simulink model "Finally_BPSK_Passband"  (R2026a)
settings: Solver=VariableStepDiscrete  StopTime=0.02  EnableMultiTasking=on
InitFcn:
  | commpassbandmodParams.Fc = 2.5e6;
  | commpassbandmodParams.F1 = commpassbandmodParams.Fc/3+.5e5;
libraries: commdigbbndpm3 x2, simulink x2, commfilt2 x2, commchan3 x1, commsink2 x1, dspsrcs4 x1, commrandsrc3 x1
Description:
  | Passband Modulation
  | 
  | This model shows a straightforward way to perform passband modulation, by multiplying a modulated complex signal with a complex sine wave to perform frequency upconversion.
settings Model: Creator=The MathWorks, Inc.  LastModifiedBy=MADHAV
settings SolverCC: InsertRTBMode=Auto
settings OptimizationCC: InitFltsAndDblsToZero=on  EfficientMapNaN2IntZero=off
settings DebuggingCC: SubsystemReferenceDiagnosticForUnitTest=warning
settings HardwareCC: ProdHWDeviceType=32-bit Generic
settings GRTTargetCC: CombineOutputUpdateFcns=off  GRTInterface=on

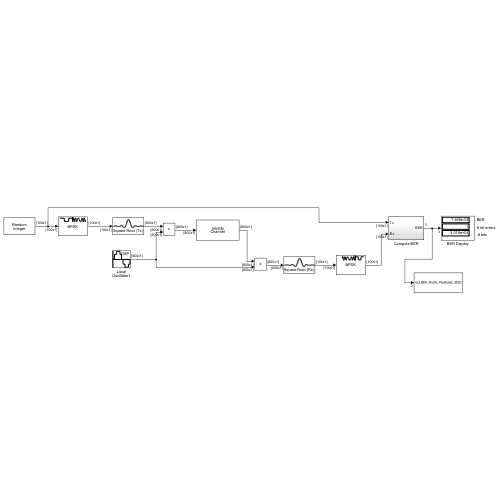
[thumbnail: Simulink's stored preview of the top-level diagram]
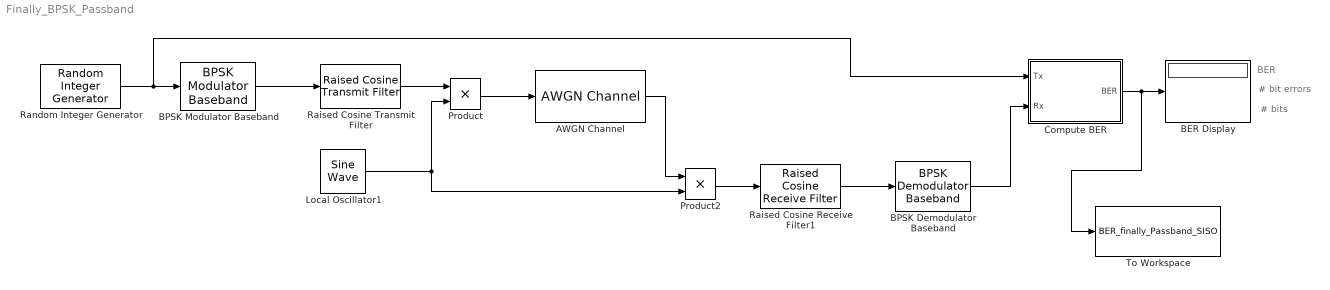
== system Finally_BPSK_Passband ==
  note: BER
  note: # bit errors
  note: # bits
  AWGN Channel : commchan3/AWGN Channel  LegacyMode=off  NoiseMethod="Signal to noise ratio  (SNR)"  noiseMode="Signal to noise ratio  (SNR)"  EbNo=10  EsNo=10  SNR=snr_variable  BitsPerSymbol=1  SignalPower=1  SpecifySymbolPeriod=off  SamplesPerSymbol=1  SymbolPeriod=1  VarianceSource=Parameter  Variance=1  RandomStream=Global stream  Seed=67  SimulateUsing=Code generation
  BER Display : Display
  BPSK Demodulator Baseband : commdigbbndpm3/BPSK Demodulator Baseband  DecType=Hard decision  VarSource=Dialog  Variance=1  Ph=0  outDtype=Inherit via internal rule  derotateFactorWordLen=16  derotateFactorDataTypeStr=Inherit: Same word length as input  derotateFactorLastDataTypeStr=Inherit: Same word length as input
      settings: LibrarySourceBlock=|
      | commhdldigbbndpm/BPSK
      | Demodulator
      | Baseband
  BPSK Modulator Baseband : commdigbbndpm3/BPSK Modulator Baseband  Ph=0  outDtype=double  outWordLen=16  outUDDataType=sfix(16)  outFracLenMode=Best precision  outFracLen=15  outDataTypeStr=double  outLastDataTypeStr=double
      settings: LibrarySourceBlock=|
      | commhdldigbbndpm/BPSK
      | Modulator
      | Baseband
  Compute BER : Subsystem
  Local Oscillator1 : dspsrcs4/Sine Wave  Amplitude=sqrt(2)  Frequency=commpassbandmodParams.Fc  Phase=0  SampleMode=Discrete  OutComplex=Real  CompMethod=Trigonometric fcn  TableSize=Speed  SampleTime=(1e-6) /8  SamplesPerFrame=800  ResetState=Restart at time zero  OutputFrames=off  dataType=double  wordLen=16  udDataType=sfix(16)  fracBitsMode=Best precision  numFracBits=15  OutDataTypeStr=double  LastOutDataTypeStr=double
  Product : Product  RndMeth=Zero
  Product2 : Product
  Raised Cosine Receive Filter1 : commfilt2/Raised Cosine Receive Filter  filtType=Square root  R=0.2  filtSpan=8  N=8  downFactor=8  downOffset=0  filterGain=2  InputProcessing=Columns as channels (frame based)  RateOptions=Enforce single-rate processing  framing=Mute  checkCoeff=off  variableName=rcRxFilt1  currentFiltSpan=10  D=5  inputOffset=0  sampMode=Mute  saveAsFlag=0  rateMode=Downsampling  checkGain=Normalized  launchFVT=on  roundingMode=Floor  overflowMode=off  coeffDataTypeStr=Inherit: Same word length as input  coeffMin=[]  coeffMax=[]  coeffLastDataTypeStr=Inherit: Same word length as input  accumDataTypeStr=Inherit: Same as product output  accumLastDataTypeStr=Inherit: Same as product output  outputDataTypeStr=Inherit: Same as accumulator  outputMin=[]  outputMax=[]  outputLastDataTypeStr=Inherit: Same as accumulator
      settings: LibrarySourceBlock=|
      | commhdlfilt/Raised Cosine
      | Receive Filter
  Raised Cosine Transmit Filter : commfilt2/Raised Cosine Transmit Filter  filtType=Square root  R=0.2  filtSpan=8  N=8  filterGain=1  InputProcessing=Columns as channels (frame based)  RateOptions=Enforce single-rate processing  framing=Mute  checkCoeff=off  variableName=rcTxFilt1  checkGain=Normalized  sampMode=Mute  saveAsFlag=0  currentFiltSpan=2*(4)  D=4  launchFVT=off  roundingMode=Floor  overflowMode=off  coeffDataTypeStr=Inherit: Same word length as input  coeffMin=[]  coeffMax=[]  coeffLastDataTypeStr=Inherit: Same word length as input  outputDataTypeStr=Inherit: Same as accumulator  outputMin=[]  outputMax=[]  outputLastDataTypeStr=Inherit: Same as accumulator
  Random Integer Generator : commrandsrc3/Random Integer Generator  SetSize=2  SeedSource=Parameter  Seed=37  SampleTime=1e-6  SamplesPerFrame=100  OutputDataType=double  SimulateUsing=Interpreted execution
  To Workspace : ToWorkspace  VariableName=BER_finally_Passband_SISO  SampleTime=-1
  wires:
  Random Integer Generator/1 -> Compute BER/1(Tx), BPSK Modulator Baseband/1
  BPSK Modulator Baseband/1 -> Raised Cosine Transmit Filter/1
  Compute BER/1(BER) -> To Workspace/1, BER Display/1
  BPSK Demodulator Baseband/1 -> Compute BER/2(Rx)
  Raised Cosine Receive Filter1/1 -> BPSK Demodulator Baseband/1
  Product2/1 -> Raised Cosine Receive Filter1/1
  Product/1 -> AWGN Channel/1
  AWGN Channel/1 -> Product2/1
  Raised Cosine Transmit Filter/1 -> Product/1
  Local Oscillator1/1 -> Product2/2, Product/2

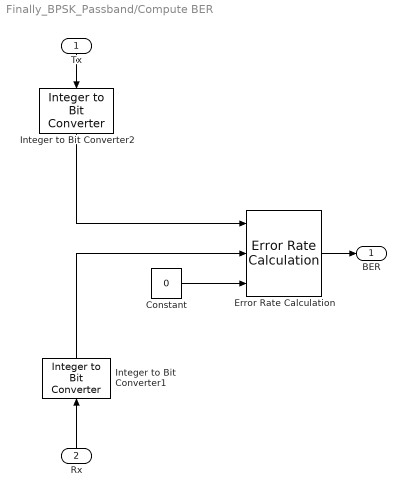
== system Finally_BPSK_Passband/Compute BER ==
  Tx : Inport
  Rx : Inport  Port=2
  Constant : Constant  Value=0  SampleTime=1e-4
  Error Rate Calculation : commsink2/Error Rate Calculation  N=16  st_delay=0  cp_mode=Entire frame  subframe=[]  PMode=Port  WsName=ErrorVec  RsMode2=on  stop=off  numErr=100  maxBits=1e6
  Integer to Bit Converter1 : simulink/Logic and Bit Operations/Integer to Bit Converter  nbits=2  signedInputValues=Unsigned  bitOrder=MSB first  outDtype=boolean
  Integer to Bit Converter2 : simulink/Logic and Bit Operations/Integer to Bit Converter  nbits=2  signedInputValues=Unsigned  bitOrder=MSB first  outDtype=boolean
  BER : Outport  VectorParamsAs1DForOutWhenUnconnected=off
  wires:
  Integer to Bit Converter2/1 -> Error Rate Calculation/1
  Integer to Bit Converter1/1 -> Error Rate Calculation/2
  Tx/1 -> Integer to Bit Converter2/1
  Error Rate Calculation/1 -> BER/1
  Rx/1 -> Integer to Bit Converter1/1
  Constant/1 -> Error Rate Calculation/3
